simulink model "rlfrequencyFPIDTune"  (R2025b)
settings: Solver=ode45  StartTime=0.0  StopTime=200  RelTol=1e-3  EnableMultiTasking=on
undefined symbols (not defined in the file): B1, B2, DBH1, DBH2, dbpu, DiscIntNeverNeededParam, GRCD1, GRCT1, GRCU1, KBESS, KD1, KDeng, Ke, Kev, KH1, KP, KP1, KP2, Kpc, KPV1, KPV2, Kr1, KT1, KW, Kw1, Kw2, N1, N2, Nev, PAGmax, PAGmin, R1, R2, Rev, T12, TBESS, Td0, Td1, Td2, Td3, Tev, TG1, Th1, Th2, TP1, TP2, Tpt1, Tpt2, TPV1, TPV2, Tr1, Trh1, Trh2, Trs1, Trs2, Tt1, TT1, Tw1, Tw2, w0
libraries: simulink x4, rllib x2, fuzblock x2
settings SolverCC: AlgebraicLoopSolver=TrustRegion  MaxZcPerStep=1.0
settings DataIOCC: LimitDataPoints=on  SaveFormat=Array  SignalLoggingName=logsOut
settings OptimizationCC: ExpressionDepthLimit=2147483647.0  InitFltsAndDblsToZero=on  LifeSpan=inf
settings DebuggingCC: SaveWithParameterizedLinksMsg=none  UnderspecifiedInitializationDetection=Classic  MergeDetectMultiDrivingBlocksExec=none  SignalResolutionControl=TryResolveAllWithWarning  MultiTaskDSMMsg=warning  FcnCallInpInsideContextMsg=warning  UnconnectedInputMsg=warning  UnconnectedOutputMsg=warning  UnconnectedLineMsg=warning  AllowSymbolicDim=off  StateNameClashWarn=warning  SFUnexpectedBacktrackingDiag=warning  SFNoUnconditionalDefaultTransitionDiag=warning  SFExecutionAtInitializationDiag=none  ArithmeticOperatorsInVariantConditions=warning
settings HardwareCC: ProdBitPerPointer=32.0  ProdBitPerSizeT=32.0  ProdBitPerPtrDiffT=32.0  ProdLargestAtomicFloat=None  ProdIntDivRoundTo=Undefined  ProdEndianess=Unspecified  ProdWordSize=32.0  ProdHWDeviceType=Specified
settings ModelReferenceCC: EnableRefExpFcnMdlSchedulingChecks=on  PropagateSignalLabelsOutOfModel=off
settings SFSimCC: SimUseLocalCustomCode=off
settings RTWCC: RTWUseLocalCustomCode=off  GPUComputeCapability=3.5  DLArmComputeVersion=19.05
settings CodeAppCC: StateflowObjectComments=on
settings GRTTargetCC: TargetFcnLib=ansi_tfl_tmw.mat  TargetLangStandard=C89/C90 (ANSI)  CombineOutputUpdateFcns=off  GRTInterface=on
settings ConfigComp: CovMetricSettings=dw  CovSaveCumulativeToWorkspaceVar=on  CovSaveSingleToWorkspaceVar=on  CovExternalEMLEnable=off

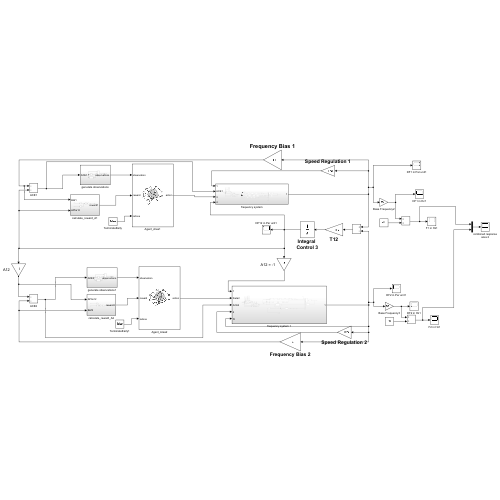
[thumbnail: Simulink's stored preview of the top-level diagram]
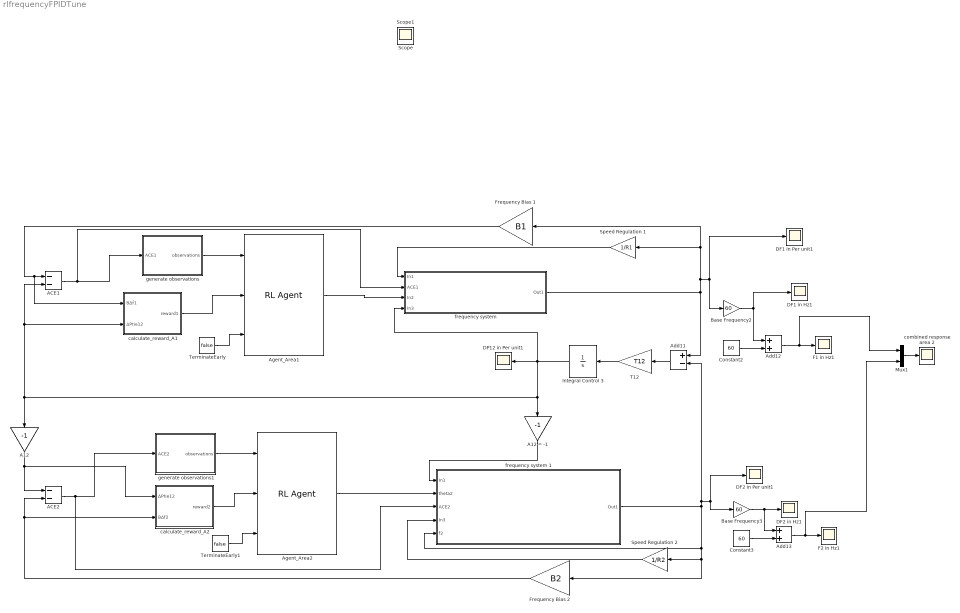
== system rlfrequencyFPIDTune ==
  A12 : Gain  Gain=-1
  A12 = -1 : Gain  Gain=-1
  ACE1 : Sum  Inputs=--
  ACE2 : Sum  Inputs=--
  Add11 : Sum  Inputs=+-
  Add12 : Sum
  Add13 : Sum
  Agent_Area1 : rllib/RL Agent  Agent=agent1  ExternalActionAsInput=off  ProvideLastAction=off  ProvideCumRwd=off  TreatAsDirectFeedthrough=on  UseStrictObservationDataTypes=off
      link override accumulate_reward/Unit Delay: InitialCondition=0
      link override accumulate_reward/cumsum/Unit Delay: InitialCondition=0
  Agent_Area2 : rllib/RL Agent  Agent=agent2  ExternalActionAsInput=off  ProvideLastAction=off  ProvideCumRwd=off  TreatAsDirectFeedthrough=on  UseStrictObservationDataTypes=off
      link override accumulate_reward/Unit Delay: InitialCondition=0
      link override accumulate_reward/cumsum/Unit Delay: InitialCondition=0
  Base Frequency2 : Gain  Gain=60
  Base Frequency3 : Gain  Gain=60
  Constant2 : Constant  Value=60
  Constant3 : Constant  Value=60
  DF1 in Hz1 : Scope
      settings: ActiveDisplayYMinimum=-0.88482  ActiveDisplayYMaximum=0.09831  DataLoggingVariableName=ScopeData12
  DF1 in Per unit1 : Scope
      settings: ActiveDisplayYMinimum=-0.01457  ActiveDisplayYMaximum=0.00367  DataLoggingVariableName=ScopeData14
  DF2 in Hz1 : Scope
      settings: ActiveDisplayYMinimum=-0.33749  ActiveDisplayYMaximum=0.0375  DataLoggingVariableName=ScopeData15
  DF2 in Per unit1 : Scope
      settings: ActiveDisplayYMinimum=-0.00562  ActiveDisplayYMaximum=0.00062  DataLoggingVariableName=ScopeData16
  DP12 in Per unit1 : Scope
      settings: ActiveDisplayYMinimum=-0.08647  ActiveDisplayYMaximum=-0.08235  DataLoggingVariableName=ScopeData18
  F1 in Hz1 : Scope
      settings: ActiveDisplayYMinimum=59.934555040014516  ActiveDisplayYMaximum=59.950342672630249  DataLoggingVariableName=ScopeData21
  F2 in Hz1 : Scope
      settings: ActiveDisplayYMinimum=59.89115  ActiveDisplayYMaximum=60.01209  DataLoggingVariableName=ScopeData22
  Frequency Bias 1 : Gain  Gain=B1
  Frequency Bias 2 : Gain  Gain=B2
  Integral Control 3 : Integrator
  Mux1 : Mux  Inputs=2
  Speed Regulation 1 : Gain  Gain=1/R1
  Speed Regulation 2 : Gain  Gain=1/R2
  T12 : Gain  Gain=T12
  TerminateEarly : Constant  Value=false
  TerminateEarly1 : Constant  Value=false
  calculate_reward_A1 : Subsystem
  calculate_reward_A2 : Subsystem
  combined response area 2 : Scope
      settings: ActiveDisplayYMinimum=59.855504382883133  ActiveDisplayYMaximum=60.059051128124558  DataLoggingVariableName=ScopeData25
  frequency system : Subsystem
  frequency system 1 : Subsystem
  generate observations : Subsystem
  generate observations1 : Subsystem
  Scope : Scope
      settings: ActiveDisplayYMinimum=-0.88405957250616218  ActiveDisplayYMaximum=11.034913762736185
  Scope1 : Scope
  wires:
  generate observations/1(observations) -> Agent_Area1/1
  calculate_reward_A1/1(reward1) -> Agent_Area1/2
  TerminateEarly/1 -> Agent_Area1/3
  Agent_Area2/1 -> frequency system 1/2(theta2)
  Constant2/1 -> Add12/2
  Agent_Area1/1 -> frequency system/3(In2)
  Frequency Bias 2/1 -> calculate_reward_A2/2(BΔf2), ACE2/2
  Add13/1 -> Mux1/2, F2 in Hz1/1
  ACE1/1 -> frequency system/2(ACE1), generate observations/1(ACE1)
  Base Frequency2/1 -> DF1 in Hz1/1, Add12/1
  Add11/1 -> T12/1
  Add12/1 -> Mux1/1, F1 in Hz1/1
  Frequency Bias 1/1 -> calculate_reward_A1/1(BΔf1), ACE1/1
  Base Frequency3/1 -> DF2 in Hz1/1, Add13/1
  Mux1/1 -> combined response area 2/1
  Constant3/1 -> Add13/2
  TerminateEarly1/1 -> Agent_Area2/3
  calculate_reward_A2/1(reward2) -> Agent_Area2/2
  generate observations1/1(observations) -> Agent_Area2/1
  ACE2/1 -> frequency system 1/3(ACE2), generate observations1/1(ACE2)
  frequency system/1(Out1) -> Add11/1, Base Frequency2/1, DF1 in Per unit1/1, Frequency Bias 1/1, Speed Regulation 1/1
  Speed Regulation 1/1 -> frequency system/1(In1)
  frequency system 1/1(Out1) -> Base Frequency3/1, DF2 in Per unit1/1, Add11/2, Frequency Bias 2/1, Speed Regulation 2/1, frequency system 1/5(f2)
  Speed Regulation 2/1 -> frequency system 1/4(In3)
  T12/1 -> Integral Control 3/1
  A12/1 -> calculate_reward_A2/1(ΔPtie12), ACE2/1
  A12 = -1/1 -> frequency system 1/1(In1)
  Integral Control 3/1 -> frequency system/4(In3), DP12 in Per unit1/1, A12 = -1/1, A12/1, calculate_reward_A1/2(ΔPtie12), ACE1/2

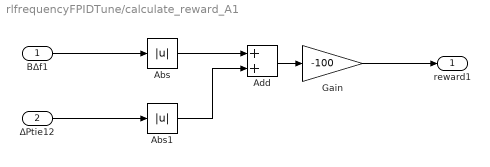
== system rlfrequencyFPIDTune/calculate_reward_A1 ==
  BΔf1 : Inport
  ΔPtie12 : Inport  Port=2
  Abs : Abs  SaturateOnIntegerOverflow=off
  Abs1 : Abs  SaturateOnIntegerOverflow=off
  Add : Sum
  Gain : Gain  Gain=-100
  reward1 : Outport  VectorParamsAs1DForOutWhenUnconnected=off
  wires:
  BΔf1/1 -> Abs/1
  Gain/1 -> reward1/1
  ΔPtie12/1 -> Abs1/1
  Abs/1 -> Add/1
  Add/1 -> Gain/1
  Abs1/1 -> Add/2

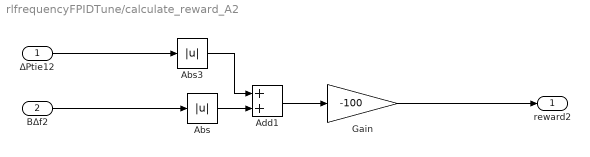
== system rlfrequencyFPIDTune/calculate_reward_A2 ==
  ΔPtie12 : Inport
  BΔf2 : Inport  Port=2
  Abs : Abs  SaturateOnIntegerOverflow=off
  Abs3 : Abs  SaturateOnIntegerOverflow=off
  Add1 : Sum
  Gain : Gain  Gain=-100
  reward2 : Outport  VectorParamsAs1DForOutWhenUnconnected=off
  wires:
  BΔf2/1 -> Abs/1
  Gain/1 -> reward2/1
  Abs/1 -> Add1/2
  ΔPtie12/1 -> Abs3/1
  Add1/1 -> Gain/1
  Abs3/1 -> Add1/1

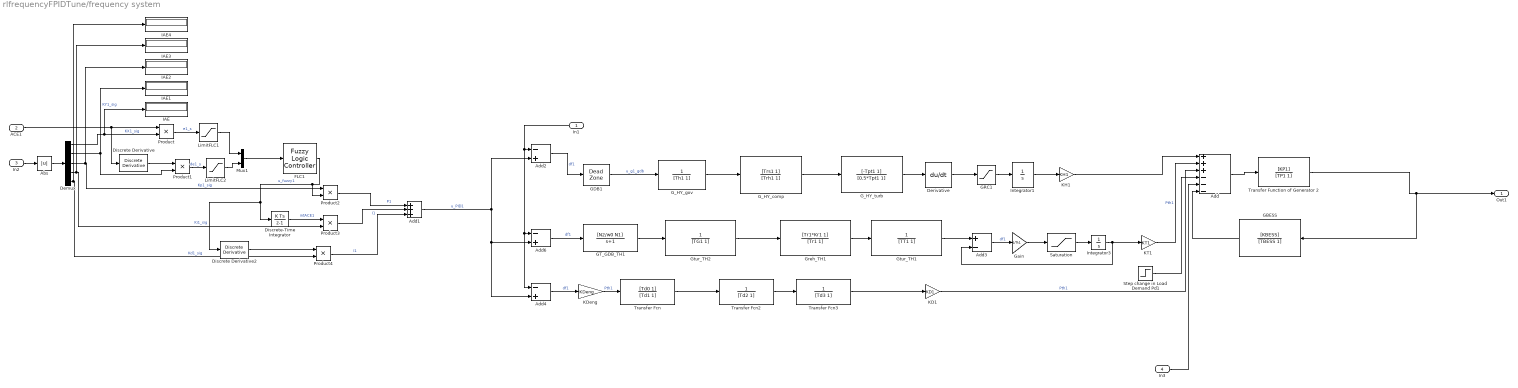
== system rlfrequencyFPIDTune/frequency system ==
  In1 : Inport
  ACE1 : Inport  Port=2
  In2 : Inport  Port=3
  In3 : Inport  Port=4
  Abs : Abs  SaturateOnIntegerOverflow=off
  Add : Sum  Inputs=+++---
  Add1 : Sum  Inputs=+++
  Add2 : Sum  Inputs=-+
  Add3 : Sum  Inputs=+-
  Add4 : Sum  Inputs=-+
  Add6 : Sum  Inputs=-+
  Demux : Demux  Outputs=5
  Derivative : Derivative
  Discrete Derivative : simulink/Discrete/Discrete Derivative  gainval=1.0  ICPrevScaledInput=0.0  OutMin=[]  OutMax=[]  OutDataType=fixdt(1, 16)  OutScaling=2^-10  DoSatur=off
  Discrete Derivative2 : simulink/Discrete/Discrete Derivative  gainval=1.0  ICPrevScaledInput=0.0  OutMin=[]  OutMax=[]  OutDataType=fixdt(1, 16)  OutScaling=2^-10  DoSatur=off
  Discrete-Time Integrator : DiscreteIntegrator  SampleTime=0.01  ICPrevOutput=DiscIntNeverNeededParam  ICPrevScaledInput=DiscIntNeverNeededParam
  FLC1 : fuzblock/Fuzzy Logic  Controller  FIS='LFC_fuzzy_trimf.fis'  OutputSampleNumber=101  DataType=double  UseLookupTable=off  NumBreakpoints=10  FuzzifiedInputs=off  RuleFiringStrengths=off  RuleOutputs=off  AggregatedOutputs=off  SimulateUsing=Interpreted execution  OutOfRangeInputValueMessage=warning  NoRuleFiredMessage=warning  EmptyOutputFuzzySetMessage=warning
  GBESS : TransferFcn  Numerator=[KBESS]  Denominator=[TBESS 1]
  GDB1 : DeadZone  LowerValue=-DBH1  UpperValue=+DBH1  ZeroCross=off
  GRC1 : Saturate  UpperLimit=GRCU1  LowerLimit=-GRCD1
  GT_GDB_TH1 : TransferFcn  Numerator=[N2/w0 N1]  Denominator=[1 1]
  G_HY_comp : TransferFcn  Numerator=[Trs1 1]  Denominator=[Trh1 1]
  G_HY_gov : TransferFcn  Numerator=1  Denominator=[Th1 1]
  G_HY_turb : TransferFcn  Numerator=[-Tpt1 1]  Denominator=[0.5*Tpt1 1]
  Gain : Gain  Gain=1/Tt1
  Greh_TH1 : TransferFcn  Numerator=[Tr1*Kr1 1]  Denominator=[Tr1 1]
  Gtur_TH1 : TransferFcn  Denominator=[TT1 1]
  Gtur_TH2 : TransferFcn  Denominator=[TG1 1]
  IAE{,1..4} (5 alike) : Display
  Integrator1 : Integrator
  Integrator3 : Integrator
  KD1 : Gain  Gain=KD1
  KDeng : Gain  Gain=KDeng
  KH1 : Gain  Gain=KH1
  KT1 : Gain  Gain=KT1
  LimitFLC1 : Saturate  UpperLimit=0.999  LowerLimit=-0.999
  LimitFLC2 : Saturate  UpperLimit=0.999  LowerLimit=-0.999
  Mux1 : Mux  Inputs=2
  Product{,1..4} (5 alike) : Product
  Saturation : Saturate  UpperLimit=GRCT1  LowerLimit=-GRCT1
  Step change in Load Demand Pd1 : Step  Time=0  Before=0.003  After=0.003  SampleTime=0
  Transfer Fcn : TransferFcn  Numerator=[Td0 1]  Denominator=[Td1 1]
  Transfer Fcn2 : TransferFcn  Denominator=[Td2 1]
  Transfer Fcn3 : TransferFcn  Denominator=[Td3 1]
  Transfer Function of Generator 2 : TransferFcn  Numerator=[KP1]  Denominator=[TP1 1]
  Out1 : Outport
  wires:
  Transfer Function of Generator 2/1 -> GBESS/1, Out1/1
  ACE1/1 -> Product/1, Discrete Derivative/1
  In2/1 -> Abs/1
  Demux/1 -> IAE/1, Product/2  "KX1_sig"
  Product/1 -> LimitFLC1/1  "e1_s"
  Discrete Derivative/1 -> Product1/1
  Demux/2 -> IAE1/1, Product1/2  "KY1_sig"
  FLC1/1 -> Discrete Derivative2/1, Discrete-Time Integrator/1, Product2/2  "u_fuzzy1"
  Discrete-Time Integrator/1 -> Product3/1  "intACE1"
  Demux/3 -> IAE2/1, Product2/1  "Kp1_sig"
  Product2/1 -> Add1/1  "P1"
  Demux/4 -> IAE3/1, Product3/2  "Ki1_sig"
  Product3/1 -> Add1/2  "I1"
  Demux/5 -> IAE4/1, Product4/2  "Kd1_sig"
  Product4/1 -> Add1/3  "I1"
  Add1/1 -> Add2/2, Add4/2, Add6/2  "u_PID1"
  GRC1/1 -> Integrator1/1
  Greh_TH1/1 -> Gtur_TH1/1
  KH1/1 -> Add/1
  Saturation/1 -> Integrator3/1
  Transfer Fcn3/1 -> KD1/1
  GBESS/1 -> Add/6
  Add2/1 -> GDB1/1  "df1"
  GDB1/1 -> G_HY_gov/1  "u_g1_gdb"
  Add4/1 -> KDeng/1  "df1"
  G_HY_turb/1 -> Derivative/1
  Integrator1/1 -> KH1/1
  Integrator3/1 -> KT1/1, Add3/2
  Gtur_TH1/1 -> Add3/1
  Transfer Fcn/1 -> Transfer Fcn2/1
  GT_GDB_TH1/1 -> Gtur_TH2/1
  Step change in Load Demand Pd1/1 -> Add/4
  Transfer Fcn2/1 -> Transfer Fcn3/1
  Gain/1 -> Saturation/1
  KD1/1 -> Add/3  "Pth1"
  In3/1 -> Add/5
  Add/1 -> Transfer Function of Generator 2/1
  G_HY_comp/1 -> G_HY_turb/1
  KDeng/1 -> Transfer Fcn/1  "Pth1"
  Derivative/1 -> GRC1/1
  Add3/1 -> Gain/1  "df1"
  G_HY_gov/1 -> G_HY_comp/1
  In1/1 -> Add4/1, Add6/1, Add2/1
  Add6/1 -> GT_GDB_TH1/1  "df1"
  KT1/1 -> Add/2  "Pth1"
  Discrete Derivative2/1 -> Product4/1
  Abs/1 -> Demux/1
  Gtur_TH2/1 -> Greh_TH1/1
  LimitFLC1/1 -> Mux1/1
  Product1/1 -> LimitFLC2/1  "de1_s"
  LimitFLC2/1 -> Mux1/2
  Mux1/1 -> FLC1/1

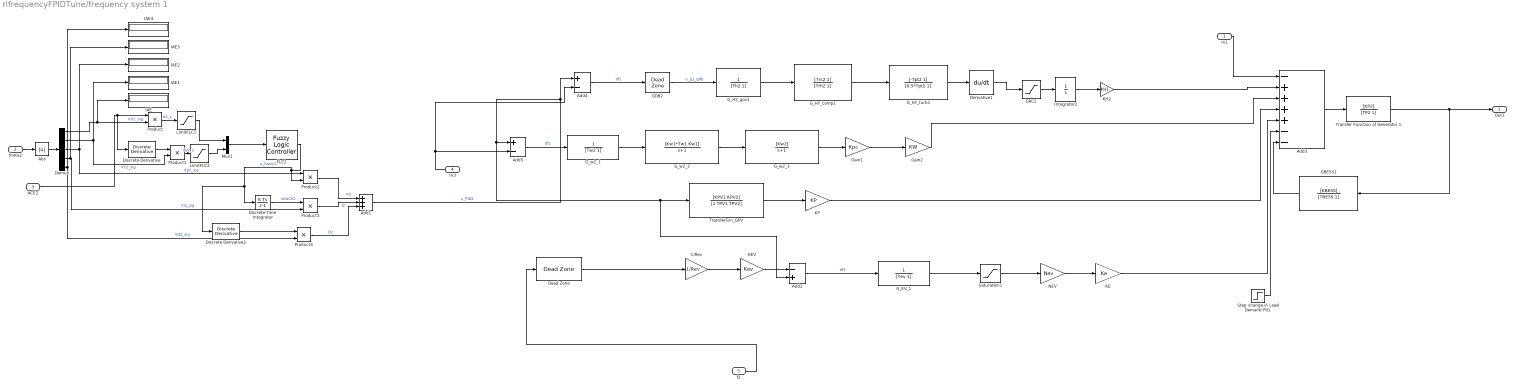
== system rlfrequencyFPIDTune/frequency system 1 ==
  In1 : Inport
  theta2 : Inport  Port=2
  ACE2 : Inport  Port=3
  In3 : Inport  Port=4
  f2 : Inport  Port=5
  1/Rev : Gain  Gain=1/Rev
  Abs : Abs  SaturateOnIntegerOverflow=off
  Add1 : Sum  Inputs=+++
  Add2 : Sum  Inputs=-+
  Add3 : Sum  Inputs=-++++--
  Add4 : Sum  Inputs=+-
  Add5 : Sum  Inputs=+-
  Dead Zone : DeadZone  LowerValue=-dbpu  UpperValue=+dbpu
  Demux : Demux  Outputs=5
  Derivative1 : Derivative
  Discrete Derivative : simulink/Discrete/Discrete Derivative  gainval=1.0  ICPrevScaledInput=0.0  OutMin=[]  OutMax=[]  OutDataType=fixdt(1, 16)  OutScaling=2^-10  DoSatur=off
  Discrete Derivative2 : simulink/Discrete/Discrete Derivative  gainval=1.0  ICPrevScaledInput=0.0  OutMin=[]  OutMax=[]  OutDataType=fixdt(1, 16)  OutScaling=2^-10  DoSatur=off
  Discrete-Time Integrator : DiscreteIntegrator  SampleTime=0.01  ICPrevOutput=DiscIntNeverNeededParam  ICPrevScaledInput=DiscIntNeverNeededParam
  FLC2 : fuzblock/Fuzzy Logic  Controller  FIS='LFC_fuzzy_trimf.fis'  OutputSampleNumber=101  DataType=double  UseLookupTable=off  NumBreakpoints=10  FuzzifiedInputs=off  RuleFiringStrengths=off  RuleOutputs=off  AggregatedOutputs=off  SimulateUsing=Interpreted execution  OutOfRangeInputValueMessage=warning  NoRuleFiredMessage=warning  EmptyOutputFuzzySetMessage=warning
  GBESS1 : TransferFcn  Numerator=[KBESS]  Denominator=[TBESS 1]
  GDB2 : DeadZone  LowerValue=-DBH2  UpperValue=+DBH2  ZeroCross=off
  GRC2 : Saturate  UpperLimit=GRCU1  LowerLimit=-GRCD1
  G_EV_1 : TransferFcn  Denominator=[Tev 1]
  G_HY_comp1 : TransferFcn  Numerator=[Trs2 1]  Denominator=[Trh2 1]
  G_HY_gov1 : TransferFcn  Numerator=1  Denominator=[Th2 1]
  G_HY_turb1 : TransferFcn  Numerator=[-Tpt2 1]  Denominator=[0.5*Tpt2 1]
  G_w2_1 : TransferFcn  Denominator=[Tw2 1]
  G_w2_2 : TransferFcn  Numerator=[Kw1*Tw1 Kw1]  Denominator=[1 1]
  G_w2_3 : TransferFcn  Numerator=[Kw2]  Denominator=[1 1]
  Gain1 : Gain  Gain=Kpc
  Gain2 : Gain  Gain=KW
  IAE{,1..4} (5 alike) : Display
  Integrator2 : Integrator
  KE : Gain  Gain=Ke
  KEV : Gain  Gain=Kev
  KH2 : Gain  Gain=KH1
  KP : Gain  Gain=KP
  LimitFLC1 : Saturate  UpperLimit=0.999  LowerLimit=-0.999
  LimitFLC2 : Saturate  UpperLimit=0.999  LowerLimit=-0.999
  Mux1 : Mux  Inputs=2
  NEV : Gain  Gain=Nev
  Product{,1..4} (5 alike) : Product
  Saturation1 : Saturate  UpperLimit=PAGmax  LowerLimit=PAGmin
  Step change in Load Demand Pd1 : Step  Time=0  Before=0.002  After=0.002  SampleTime=0
  Transfer Function of Generator 1 : TransferFcn  Numerator=[KP2]  Denominator=[TP2 1]
  TransferFcn_GPV : TransferFcn  Numerator=[KPV1 KPV2]  Denominator=[1 TPV1 TPV2]
  Out1 : Outport
  wires:
  Product2/1 -> Add1/1  "P2"
  Demux/4 -> IAE3/1, Product3/2  "Ki2_sig"
  Discrete-Time Integrator/1 -> Product3/1  "intACE2"
  Add1/1 -> Add4/1, Add2/2, TransferFcn_GPV/1, Add5/1  "u_PID2"
  ACE2/1 -> Product/1, Discrete Derivative/1
  Product3/1 -> Add1/2  "I2"
  Demux/1 -> IAE/1, Product/2  "KX2_sig"
  theta2/1 -> Abs/1
  Demux/2 -> IAE1/1, Product1/2  "KY2_sig"
  Demux/5 -> Product4/2, IAE4/1  "Kd2_sig"
  FLC2/1 -> Discrete Derivative2/1, Discrete-Time Integrator/1, Product2/2  "u_fuzzy2"
  Product4/1 -> Add1/3  "D2"
  Discrete Derivative/1 -> Product1/1
  Product/1 -> LimitFLC1/1  "e2_s"
  Demux/3 -> Product2/1, IAE2/1  "Kp2_sig"
  Transfer Function of Generator 1/1 -> GBESS1/1, Out1/1
  Derivative1/1 -> GRC2/1
  f2/1 -> Dead Zone/1
  Add3/1 -> Transfer Function of Generator 1/1
  Add2/1 -> G_EV_1/1  "df1"
  Saturation1/1 -> NEV/1
  KH2/1 -> Add3/2
  G_HY_turb1/1 -> Derivative1/1
  G_w2_1/1 -> G_w2_2/1
  G_w2_2/1 -> G_w2_3/1
  G_EV_1/1 -> Saturation1/1
  G_w2_3/1 -> Gain1/1
  KP/1 -> Add3/4
  GDB2/1 -> G_HY_gov1/1  "u_g1_gdb"
  TransferFcn_GPV/1 -> KP/1
  In3/1 -> Add5/2, Add4/2
  KEV/1 -> Add2/1
  G_HY_gov1/1 -> G_HY_comp1/1
  Step change in Load Demand Pd1/1 -> Add3/6
  Gain2/1 -> Add3/3
  In1/1 -> Add3/1
  Add4/1 -> GDB2/1  "df1"
  G_HY_comp1/1 -> G_HY_turb1/1
  KE/1 -> Add3/5
  NEV/1 -> KE/1
  Gain1/1 -> Gain2/1
  Add5/1 -> G_w2_1/1  "df1"
  1/Rev/1 -> KEV/1
  GRC2/1 -> Integrator2/1
  Dead Zone/1 -> 1/Rev/1
  Integrator2/1 -> KH2/1
  GBESS1/1 -> Add3/7
  Discrete Derivative2/1 -> Product4/1
  Abs/1 -> Demux/1
  LimitFLC1/1 -> Mux1/1
  Product1/1 -> LimitFLC2/1  "de2_s"
  LimitFLC2/1 -> Mux1/2
  Mux1/1 -> FLC2/1

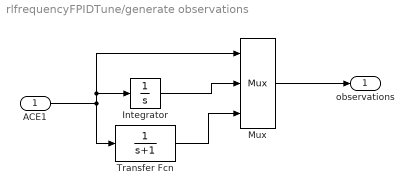
== system rlfrequencyFPIDTune/generate observations ==
  ACE1 : Inport
  Integrator : Integrator
  Mux : Mux  Inputs=3
  Transfer Fcn : TransferFcn  Denominator=[1 1]
  observations : Outport  VectorParamsAs1DForOutWhenUnconnected=off
  wires:
  ACE1/1 -> Transfer Fcn/1, Integrator/1, Mux/1
  Mux/1 -> observations/1
  Transfer Fcn/1 -> Mux/3
  Integrator/1 -> Mux/2

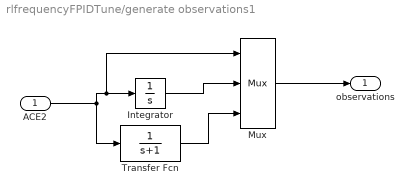
== system rlfrequencyFPIDTune/generate observations1 ==
  ACE2 : Inport
  Integrator : Integrator
  Mux : Mux  Inputs=3
  Transfer Fcn : TransferFcn  Denominator=[1 1]
  observations : Outport  VectorParamsAs1DForOutWhenUnconnected=off
  wires:
  ACE2/1 -> Transfer Fcn/1, Integrator/1, Mux/1
  Mux/1 -> observations/1
  Transfer Fcn/1 -> Mux/3
  Integrator/1 -> Mux/2
